simulink model "soc_01_coulomb_counting"  (R2025a)
settings: Solver=FixedStepDiscrete  StartTime=0.0  StopTime=240  FixedStep=1  RelTol=1e-3
undefined symbols (not defined in the file): DiscIntNeverNeededParam
Description:
  | Lesson 1: Coulomb counting for a simulated 2 Ah battery. The reference and estimate receive the same current but start at 80% and 50%. Open Compare SOC and run. Try changing the estimated initial condition to 80%.
settings Model: Creator=mosri  LastModifiedBy=mosri

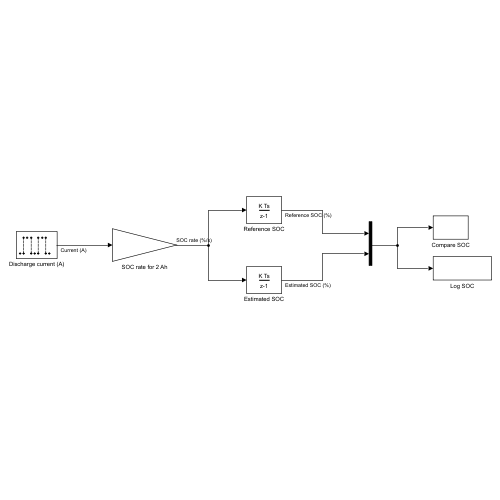
[thumbnail: Simulink's stored preview of the top-level diagram]
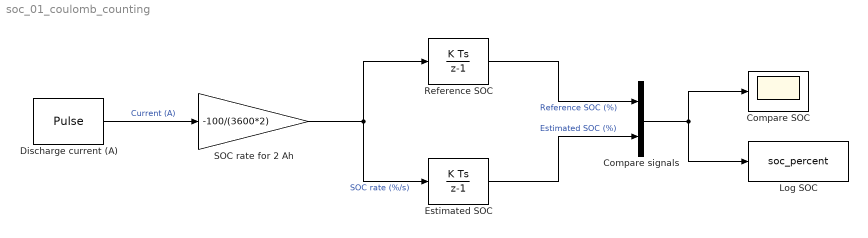
== system soc_01_coulomb_counting ==
  Compare SOC : Scope
      settings: Title=Coulomb counting: reference vs. estimate  ActiveDisplayYMinimum=45  ActiveDisplayYMaximum=85  YLabel=SOC (%)
  Compare signals : Mux  Inputs=2
  Discharge current (A) : DiscretePulseGenerator  Period=120  PulseWidth=60
  Estimated SOC : DiscreteIntegrator  InitialCondition=50  ICPrevOutput=DiscIntNeverNeededParam  ICPrevScaledInput=DiscIntNeverNeededParam
  Log SOC : ToWorkspace  VariableName=soc_percent  SampleTime=-1
  Reference SOC : DiscreteIntegrator  InitialCondition=80  ICPrevOutput=DiscIntNeverNeededParam  ICPrevScaledInput=DiscIntNeverNeededParam
  SOC rate for 2 Ah : Gain  Gain=-100/(3600*2)
  wires:
  Discharge current (A)/1 -> SOC rate for 2 Ah/1  "Current (A)"
  SOC rate for 2 Ah/1 -> Reference SOC/1, Estimated SOC/1  "SOC rate (%/s)"
  Reference SOC/1 -> Compare signals/1  "Reference SOC (%)"
  Estimated SOC/1 -> Compare signals/2  "Estimated SOC (%)"
  Compare signals/1 -> Compare SOC/1, Log SOC/1
